simulink model "oc4_VarMass"  (R2026a)
settings: Solver=ode4  StartTime=0  StopTime=400  FixedStep=0.1  MaxStep=0.1  EnableMultiTasking=on
values from neighbouring files (symbols this model uses):
  simu = simulationClass()    [wecSimInputFile.m]
  waves = waveClass('regular')    [wecSimInputFile.m]
undefined symbols (not defined in the file or in its folder): body, constraint, X, Y, Z
libraries: nesl_utility x22, sm_lib x12, WECSim_Lib_Body_Elements x4, vrlib x1, matrix_library x1, WECSim_Lib_Constraints x1, WECSim_Lib_Frames x1
(part 2 of 3)

== system oc4_VarMass/Float/Hydrodynamic Body/Variable Hydrodynamics Control ==
  note: Developer note: When creating a new bus selector, it will only show the variables within hydroForce if they already exist in the workspace, which is inconventient. Copy this bus selector to more easily add calls to variables from hydroForce. This bus selector should already contains all variables in hydroForce which can then be selected, and extras deleted.
      |
      | Alternatively, open the bus selector block and use programmatic commands to set the output variables, e.g.
      | >> set_param(gcb, 'OutputSignals', 'storage.mass, volume');
  Bus Selector : BusSelector  Commented=on  OutputSignals=linearHydroRestCoef,storage,quadDrag,linearDamping,fExt,fExt.re,fExt.im,fExt.md,fAddedMass,fDamping,irkb,storage.mass,storage.inertia,storage.inertiaProducts,storage.fAddedMass,userDefinedFe,totDOF,fExt.dofGrd,fExt.dirGrd,fExt.wGrd,fExt.fEHRE,fExt.fEHIM,fExt.fEHMD
  Constant : Constant  Value=body.hydroForce  VectorParams1D=off  OutDataTypeStr=Bus: bus_body1_hydroForce
  From : From  Commented=on  GotoTag=body1_hydroForce
  Variable Hydrodynamics Subsystem : Subsystem  Variant=on  VariantControl=sv_b1_variableHydro  mask{body=body}
  tag scope: body1_hydroForce=global
  wires:
  From/1 -> Bus Selector/1
  Variable Hydrodynamics Subsystem/1(selected_hydroForce) -> [body1_hydroForce]
  Constant/1 -> Variable Hydrodynamics Subsystem/1(all_hydroForce)

== system oc4_VarMass/Float/Hydrodynamic Body/Wave Diffraction and Excitation Force Calculation ==
  note: The excitation force = F_wave * ramp function
  Time : Inport
  Displacement : Inport  Port=2
  WaveElv : Inport  Port=3
  Add : Sum  Inputs=+++
  Constant : Constant
  FexcInputs : Subsystem
  Less Than : RelationalOperator  Operator=<  OutDataTypeStr=boolean  RndMeth=Simplest  InputSameDT=off
  Linear Wave Excitation Force Variant Subsystem : Subsystem  Variant=on  VariantControl=sv_irregularWavesNonLinYaw_b1  mask{Nwave=waves(1)}
      mask prompts: Nwave "Wave Instance"
  Nonlinear FK Force Variant Subsystem : Subsystem  Variant=on
  Product : Product
  Ramp Function Time : Constant  Value=simu.rampTime
  Ramp function : Subsystem
  Second Order Excitation Force Variant Subsystem : Subsystem  Variant=on
  Switch : Switch  Criteria=u2 ~= 0  SaturateOnIntegerOverflow=off  InputSameDT=off
  F_Excitation : Outport  PortDimensions=body.dof
  wires:
  [body1_hydroForce] -> FexcInputs/4(body_hydroForce)
  FexcInputs/4(Out4) -> Second Order Excitation Force Variant Subsystem/2(body_hydroForce), Linear Wave Excitation Force Variant Subsystem/3(body_hydroForce)
  Second Order Excitation Force Variant Subsystem/1(Second Order Excitation) -> Add/3
  FexcInputs/1(Out1) -> Nonlinear FK Force Variant Subsystem/1(Time), Less Than/1, Ramp function/1(Time), Linear Wave Excitation Force Variant Subsystem/1(Time), Second Order Excitation Force Variant Subsystem/1(Time)
  FexcInputs/3(Out3) -> Nonlinear FK Force Variant Subsystem/3(WaveElv)
  WaveElv/1 -> FexcInputs/3(WaveElv)
  Displacement/1 -> FexcInputs/2(Displacement)
  Time/1 -> FexcInputs/1(Time)
  FexcInputs/2(Out2) -> Nonlinear FK Force Variant Subsystem/2(Displacement), Second Order Excitation Force Variant Subsystem/3(displacement), Linear Wave Excitation Force Variant Subsystem/2(Displacement)
  Constant/1 -> Switch/3
  Less Than/1 -> Switch/2
  Ramp function/1(R) -> Switch/1
  Ramp Function Time/1 -> Less Than/2
  Nonlinear FK Force Variant Subsystem/1(Nonlinear Excitation) -> Add/2
  Linear Wave Excitation Force Variant Subsystem/1(Linear Excitation) -> Add/1
  Product/1 -> F_Excitation/1  "F_Excitation"
  Add/1 -> Product/2  "F_wave"
  Switch/1 -> Product/1  "R"

== system oc4_VarMass/Float/Hydrodynamic Body/Wave Radiation Forces Calculation ==
  note: F_AddedMass = AM * a
  Velocity : Inport
  Acceleration : Inport  Port=2
  Bus Selector : BusSelector  OutputSignals=fAddedMass
  Product1 : Product  Multiplication=Matrix(*)
  SS CI and Constant-Damping-CoeVariant Subsystem : Subsystem  Variant=on
  F_RadiationDamping : Outport
  F_AddedMass : Outport  Port=2
  wires:
  Bus Selector/1 -> Product1/1  "<fAddedMass>"
  [body1_hydroForce] -> Bus Selector/1
  Acceleration/1 -> Product1/2
  SS CI and Constant-Damping-CoeVariant Subsystem/1(Out1) -> F_RadiationDamping/1  "F_RadiationDamping"
  Velocity/1 -> SS CI and Constant-Damping-CoeVariant Subsystem/1(velocity)
  Product1/1 -> F_AddedMass/1  "F_AddedMass"

== system oc4_VarMass/Float/Hydrodynamic Body/Yaw Force Transforms ==
  F_Excitation : Inport
  F_RadiationDamping : Inport  Port=2
  In2 : Inport  Port=3
  F_AddedMass : Inport  Port=4
  F_Restoring : Inport  Port=5
  Constant : Constant  Value=body.yaw.option
  Yaw Force Transforms : MATLAB Function  TreatAsAtomicUnit=on
  Out1 : Outport
  Out2 : Outport  Port=2
  Out3 : Outport  Port=3
  Out4 : Outport  Port=4
  wires:
  Yaw Force Transforms/1(F_Excitation) -> Out1/1
  Yaw Force Transforms/3(F_AddedMass) -> Out3/1
  Yaw Force Transforms/2(F_RadiationDamping) -> Out2/1
  F_RadiationDamping/1 -> Yaw Force Transforms/2(dispGlobal)
  F_AddedMass/1 -> Yaw Force Transforms/4(F_AddedMassLocal)
  Yaw Force Transforms/4(F_Restoring) -> Out4/1
  F_Excitation/1 -> Yaw Force Transforms/5(F_ExcitationLocal)
  In2/1 -> Yaw Force Transforms/3(F_RadiationDampingLocal)
  F_Restoring/1 -> Yaw Force Transforms/6(F_RestoringLocal)
  Constant/1 -> Yaw Force Transforms/1(yaw)

== system oc4_VarMass/Float/Hydrodynamic Body/Yaw Kinematic Transforms ==
  note: If simu.b2b == 0, no body to body interaction is used (noB2B)
      | If simu.b2b == 1, use body to body interaction (B2B)
  note: 1) Add Subsystem or Model blocks as valid variant choices.
      | 2) You cannot connect blocks at this level. At simulation, connectivity is automatically
      | determined, based on the active variant and port name matching.
  dispGlobal : Inport
  velGlobal : Inport  Port=2
  accGlobal : Inport  Port=3
  No B2B : Subsystem  VariantControl=sv_noB2B
  With B2B : Subsystem  VariantControl=sv_B2B
  dispLoc : Outport
  velLoc : Outport  Port=2
  accLoc : Outport  Port=3

== system oc4_VarMass/Float/Hydrodynamic Body/B2B Subsystem/B2B ==
  CrossCoupling : Subsystem  mask{body=body}
      mask prompts: body "Body Number"
      mask help: This is used to
      mask init:
      | %In the initialization tab we place the code modifying the block
      | 
      | cb = gcb;
      | % position of initial blocks
      | set_param([cb '/vel1'],'Position',[200 1*50 240 (1*50+30)])
      | set_param([cb '/Mux1'], 'Position',[375 40 380 90])
      | set_param([cb '/vel'], 'Position',[410 59 440 71])
      | set_param([cb '/acc1'],'Position',[600 1*50 640 (1*50+30)])
      | set_param([cb '/Mux2'], 'Position',[775 40 780 90])
      | set_param([cb '/acc'], 'Position',[810 59 840 71])
      | set_param([cb '/Transport Delay1'], 'Position', [650 1*50 690 (1*50+30)])
      | 
      | % add/delete lines & blocks
      | newInputs = 0;
      | numbodies = body.total;
      | iBod = 2;
      | while iBod < 100
      |     try 
      |         find_system([cb,'/vel',num2str(iBod)],'Type','Block');
      |         if iBod > numbodies
      |             %delete 'From' blocks and lines if bodynumber > total bodies
      |             delete_line(cb,['vel',num2str(iBod),'/1'],['Mux',num2str(1),'/',num2str(iBod)])
      |             delete_line(cb,['acc',num2str(iBod),'/1'],['Transport Delay',num2str(iBod),'/1'])
      |             delete_line(cb,['Transport Delay',num2str(iBod),'/1'],['Mux',num2str(2),'/',num2str(iBod)])
      |             delete_block([cb '/vel',num2str(iBod)])
      |             delete_block([cb '/acc',num2str(iBod)])
      |             delete_block([cb '/Transport Delay',num2str(iBod)])
      |         end
      |     catch
      |         %set number of outputs for 'Mux Creator' blocks 
      |         if newInputs==0
      |             set_param([cb,'/Mux1'],'Inputs',num2str(numbodies))
      |             set_param([cb,'/Mux2'],'Inputs',num2str(numbodies))
      |         end
      |         if iBod <= numbodies
      |             newInputs = newInputs + 1;
      |             %add velocity 'From' block
      |             add_block('simulink/Signal Routing/From', [cb,'/vel',num2str(iBod)],'MakeNameUnique', 'on',...
      |             'Position',[200 iBod*50 240 (iBod*50+30)], 'BackgroundColor','green')
      |             h=[cb,'/vel',num2str(iBod)];
      |             responseName=['vel' num2str(iBod)];
      |             set_param(h,'GotoTag',responseName);
      |             %add acceleration 'From' block
      |             add_block('simulink/Signal Routing/From', [cb,'/acc',num2str(iBod)],'MakeNameUnique', 'on',...
      |             'Position',[600 iBod*50 640 (iBod*50+30)], 'BackgroundColor','green')
      |             h=[cb,'/acc',num2str(iBod)];
      |             responseName=['acc' num2str(iBod)];
      |             set_param(h,'GotoTag',responseName);
      |             % add transport delay block 
      |             add_block('simulink/Continuous/Transport Delay', [cb,'/Transport Delay',num2str(iBod)],'MakeNameUnique', 'on',...
      |             'Position',[650 iBod*50 690 (iBod*50+30)])
      |             h=[cb,'/Transport Delay',num2str(iBod)];
      |             set_param(h,'DelayTime',num2str(10e-8));
      |             %add lines
      |             add_line(cb,['vel',num2str(iBod),'/1'],['Mux',num2str(1),'/',num2str(iBod)])
      |             add_line(cb,['acc',num2str(iBod),'/1'],['Transport Delay',num2str(iBod),'/1'])
      |             add_line(cb,['Transport Delay',num2str(iBod),'/1'],['Mux',num2str(2),'/',num2str(iBod)])
      |             
      |         else
      |             break
      |         end
      |     end
      |     iBod = iBod + 1;
      | end
      mask Callback body: %customsat_callback('input',gcb)
      mask DialogControl DescGroupVar Prompt: Coupling Block
      mask DialogControl DescTextVar Prompt: This block transfers the velocity and acceleration vectors between bodies allowing for the coupled hydrodynamic forces to be calculated.  This block should not be included if there is only one body or if the hydrodynamic coupling parameter is set to 'No' in the rigid body block.
  vel : Outport
  acc : Outport  Port=2
  wires:
  CrossCoupling/2(acc) -> acc/1
  CrossCoupling/1(vel) -> vel/1

== system oc4_VarMass/Float/Hydrodynamic Body/B2B Subsystem/noB2B ==
  vel_in : Inport
  acc_in : Inport  Port=2
  vel : Outport
  acc : Outport  Port=2
  wires:
  acc_in/1 -> acc/1
  vel_in/1 -> vel/1  "x"

== system oc4_VarMass/Float/Hydrodynamic Body/Hydrostatic Restoring Force Calculation/Linear and Nonlinear Restoring Force Variant Subsystem ==
  note: 1) Add Subsystem or Model blocks as valid variant choices.
      | 2) You cannot connect blocks at this level. At simulation, connectivity is automatically
      | determined, based on the active variant and port name matching.
  note: If simu.nlHydro == 0, use the linear force option.
      | If simu.nlHydro > 0, use the nonlinear force option.
  In1 : Inport
  In2 : Inport  Port=2
  Linear Hydrostatic Restoring Force : Subsystem  VariantControl=sv_b1_linearHydro
  Nonlinear Hydrostatic Restoring Force : Subsystem  VariantControl=sv_b1_nonlinearHydro
  Out1 : Outport

== system oc4_VarMass/Float/Hydrodynamic Body/Morison Element and Viscous Damping Force Calculation/Morison Element Variant Subsystem ==
  note: 1) Add Subsystem or Model blocks as valid variant choices.
      | 2) You cannot connect blocks at this level. At simulation, connectivity is automatically
      | determined, based on the active variant and port name matching.
  note: If body.morisonElement.option == 0, Morison element is off and the Morison force is 0
      | If body.morisonElement.option == 1 | 2, Morison element is on
  displacement : Inport
  velocity : Inport  Port=2
  acceleration : Inport  Port=3
  time : Inport  Port=4
  Morison Element Off : Subsystem  VariantControl=sv_b1_MEOff
  Morison Element On : Subsystem  Variant=on  VariantControl=sv_b1_MEOn
  morison_force : Outport

== system oc4_VarMass/Float/Hydrodynamic Body/Nonlinear Wave Elevation/Linear or Instantaneous Free Surface ==
  note: 1) Add Subsystem or Model blocks as valid variant choices.
      | 2) You cannot connect blocks at this level. At simulation, connectivity is automatically
      | determined, based on the active variant and port name matching.
  note: If simu.nlHydro < 2, use the mean water free surface.
      | If simu.nlHydro == 2, use the instantaneous water free surface
  In1 : Inport
  In2 : Inport  Port=2
  Instantaneous Water Free Surface : Subsystem  VariantControl=sv_b1_instFS
  Mean Water Free Surface : Subsystem  VariantControl=sv_b1_meanFS
  Out1 : Outport

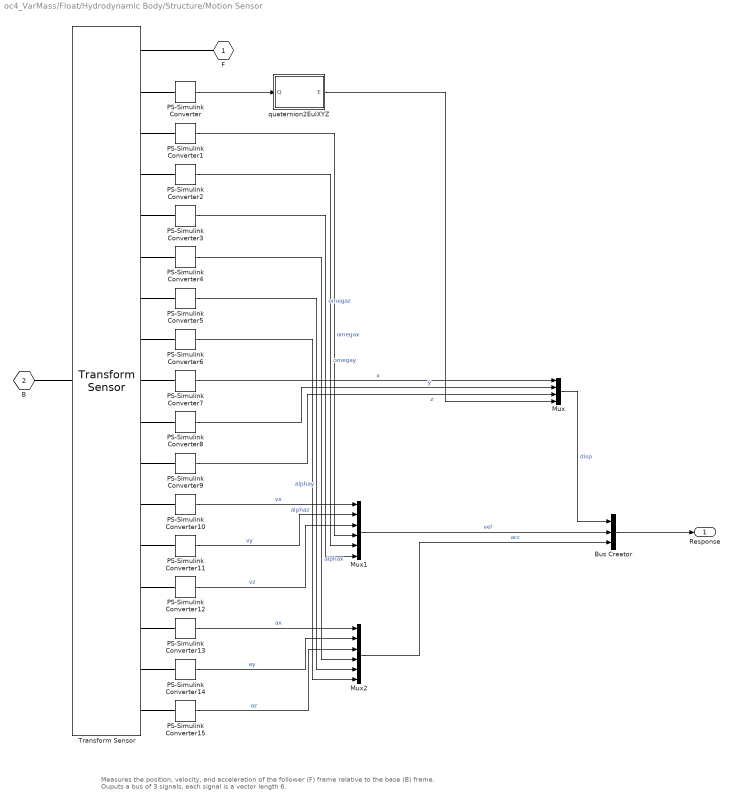
== system oc4_VarMass/Float/Hydrodynamic Body/Structure/Motion Sensor ==
  note: Measures the position, velocity, and acceleration of the follower (F) frame relative to the base (B) frame.
      | Ouputs a bus of 3 signals, each signal is a vector length 6.
  Bus Creator : BusCreator  Inputs=3
  Mux : Mux
  Mux1 : Mux  Inputs=6
  Mux2 : Mux  Inputs=6
  PS-Simulink Converter{,1..15} (16 alike) : nesl_utility/PS-Simulink Converter  PhysicalDomain=network_engine_domain  SubClassName=ps_output  LeftPortType=input  RightPortType=output  PseudoPeriodic=off  Frequencies=[]  VectorFormat=1-D array  Unit=1  AffineConversion=off
  Transform Sensor : sm_lib/Frames and Transforms/Transform Sensor  MeasurementFrame=World  RotationSequence=XYX  SenseAngle=off  SenseAxis=off  SenseQ=on  SenseR=off  SenseRotationSequence=off  SenseOmegaX=on  SenseOmegaY=on  SenseOmegaZ=on  SenseOmega=off  SenseQDot=off  SenseRDot=off  SenseRotationSequenceDot=off  SenseAlphaX=on  SenseAlphaY=on  SenseAlphaZ=on  SenseAlpha=off  SenseQDDot=off  SenseRDDot=off  SenseX=on  SenseY=on  SenseZ=on  SenseXYZ=off  SenseRad=off  SenseAzim=off  SenseDist=off  SenseInc=off  SenseXDot=on  SenseYDot=on  SenseZDot=on  SenseXYZDot=off  SenseRadDot=off  SenseAzimDot=off  SenseDistDot=off  SenseIncDot=off  SenseXDDot=on  SenseYDDot=on  SenseZDDot=on  SenseXYZDDot=off  SenseRadDDot=off  SenseAzimDDot=off  SenseDistDDot=off  SenseIncDDot=off
  quaternion2EulXYZ : MATLAB Function  TreatAsAtomicUnit=on
  F : PMIOPort  Side=Right
  B : PMIOPort  Port=2  Side=Left
  Response : Outport
  wires:
  PS-Simulink Converter/1 -> quaternion2EulXYZ/1(Q)
  quaternion2EulXYZ/1(E) -> Mux/4
  PS-Simulink Converter4/1 -> Mux2/4  "alphax"
  PS-Simulink Converter10/1 -> Mux1/1  "vx"
  PS-Simulink Converter12/1 -> Mux1/3  "vz"
  PS-Simulink Converter13/1 -> Mux2/1  "ax"
  PS-Simulink Converter14/1 -> Mux2/2  "ay"
  Mux/1 -> Bus Creator/1  "disp"
  Mux1/1 -> Bus Creator/2  "vel"
  Mux2/1 -> Bus Creator/3  "acc"
  PS-Simulink Converter7/1 -> Mux/1  "x"
  PS-Simulink Converter8/1 -> Mux/2  "y"
  PS-Simulink Converter9/1 -> Mux/3  "z"
  PS-Simulink Converter5/1 -> Mux2/5  "alphay"
  PS-Simulink Converter6/1 -> Mux2/6  "alphaz"
  PS-Simulink Converter1/1 -> Mux1/4  "omegax"
  PS-Simulink Converter2/1 -> Mux1/5  "omegay"
  PS-Simulink Converter11/1 -> Mux1/2  "vy"
  PS-Simulink Converter3/1 -> Mux1/6  "omegaz"
  PS-Simulink Converter15/1 -> Mux2/3  "az"
  Bus Creator/1 -> Response/1
  connections:
  Transform Sensor/RConn16 -- PS-Simulink Converter14/LConn1
  PS-Simulink Converter13/LConn1 -- Transform Sensor/RConn15
  PS-Simulink Converter12/LConn1 -- Transform Sensor/RConn14
  Transform Sensor/RConn13 -- PS-Simulink Converter11/LConn1
  PS-Simulink Converter10/LConn1 -- Transform Sensor/RConn12
  PS-Simulink Converter9/LConn1 -- Transform Sensor/RConn11
  Transform Sensor/RConn10 -- PS-Simulink Converter8/LConn1
  PS-Simulink Converter7/LConn1 -- Transform Sensor/RConn9
  Transform Sensor/RConn8 -- PS-Simulink Converter6/LConn1
  PS-Simulink Converter5/LConn1 -- Transform Sensor/RConn7
  Transform Sensor/RConn6 -- PS-Simulink Converter4/LConn1
  PS-Simulink Converter3/LConn1 -- Transform Sensor/RConn5
  Transform Sensor/RConn4 -- PS-Simulink Converter2/LConn1
  PS-Simulink Converter1/LConn1 -- Transform Sensor/RConn3
  Transform Sensor/RConn2 -- PS-Simulink Converter/LConn1
  PS-Simulink Converter15/LConn1 -- Transform Sensor/RConn17
  Transform Sensor/RConn1 -- F/RConn1
  B/RConn1 -- Transform Sensor/LConn1

== system oc4_VarMass/Float/Hydrodynamic Body/Variable Hydrodynamics Control/Variable Hydrodynamics Subsystem ==
  note: 1) Add Subsystem or Model blocks as valid variant choices.
      | 2) You cannot connect blocks at this level. At simulation, connectivity is automatically
      | determined, based on the active variant and port name matching.
  all_hydroForce : Inport
  noVariableHydro : Subsystem  VariantControl=sv_b1_noVariableHydro
  variableHydro : Subsystem  VariantControl=sv_b1_variableHydro  mask{body=body}
      mask prompts: body "Body Number:"
      mask init:
      | hydroForceElements = fields(body.hydroForce);
      | 
      | nElements = length(hydroForceElements);
      | elementString = hydroForceElements{1};
      | if nElements > 1
      |     for i=2:nElements
      |         elementString = [elementString ', ' hydroForceElements{i}]; 
      |     end
      | end
      | 
      | % Update bus signals with the name of hydroForce elements (hf1, hf2, etc)
      | h = [gcb '/Bus Selector'];
      | set_param(h, 'OutputSignals', elementString);
      | 
      | % Update number of switch inputs
      | h = [gcb '/Multiport Switch'];
      | set_param(h, 'Inputs', num2str(nElements));
      | 
      | % Connect bus outputs and switch inputs
      | for i = 1:nElements
      |     try
      |         add_line(gcb, ...
      |             ['Bus Selector/' num2str(i)], ...
      |             ['Multiport Switch/' num2str(i+1)],...
      |             'autorouting','on');
      |     catch
      |     end
      | end
      | 
      | % Connect the initial case (default hydroForce) to the end of the multiport switch (default case)
      | hydroForceIndexInitial = body.variableHydro.hydroForceIndexInitial;
      | try
      |     add_line(gcb, ...
      |         ['Bus Selector/' num2str(hydroForceIndexInitial)], ...
      |         ['Multiport Switch/' num2str(nElements+2)],...
      |         'autorouting','on');
      | catch
      | end
  selected_hydroForce : Outport

== system oc4_VarMass/Float/Hydrodynamic Body/Wave Diffraction and Excitation Force Calculation/FexcInputs ==
  Time : Inport
  Displacement : Inport  Port=2
  WaveElv : Inport  Port=3
  body_hydroForce : Inport  Port=4
  Out1 : Outport
  Out2 : Outport  Port=2
  Out3 : Outport  Port=3
  Out4 : Outport  Port=4
  wires:
  body_hydroForce/1 -> Out4/1
  Displacement/1 -> Out2/1
  Time/1 -> Out1/1
  WaveElv/1 -> Out3/1

== system oc4_VarMass/Float/Hydrodynamic Body/Wave Diffraction and Excitation Force Calculation/Linear Wave Excitation Force Variant Subsystem ==
  note: 1) Add Subsystem or Model blocks as valid variant choices.
      | 2) You cannot connect blocks at this level. At simulation, connectivity is automatically
      | determined, based on the active variant and port name matching.
  note: No wave includes wave.type == 'noWave' or 'noWaveCIC'
      | Regular wave includes wave.type == 'regular' or 'regularCIC'
      | Irregular wave includes wave.type == 'irregular' or 'spectrumImport'
  Time : Inport
  Displacement : Inport  Port=2
  body_hydroForce : Inport  Port=3
  Irregular Wave Excitation Force : Subsystem  VariantControl=sv_irregularWaves_b1
  Irregular Wave NonLinearYaw : Subsystem  VariantControl=sv_irregularWavesYaw_b1
  Irregular Wave Full Direction : Subsystem  VariantControl=sv_fullDirIrregularWaves_b1
  No Wave Excitation Force : Subsystem  VariantControl=sv_noWave
  Regular Wave Excitation Force : Subsystem  VariantControl=sv_regularWaves_b1
  Regular Wave NonLinear Yaw : Subsystem  VariantControl=sv_regularWavesYaw_b1
  User Defined Wave Excitation Force : Subsystem  VariantControl=sv_udfWaves
  Linear Excitation : Outport

== system oc4_VarMass/Float/Hydrodynamic Body/Wave Diffraction and Excitation Force Calculation/Nonlinear FK Force Variant Subsystem ==
  note: 1) Add Subsystem or Model blocks as valid variant choices.
      | 2) You cannot connect blocks at this level. At simulation, connectivity is automatically
      | determined, based on the active variant and port name matching.
  note: If simu.nlHydro == 0, use No Nonlinear FroudeKrylov force option (nonlinear force is zero),
      | If simu.nlHydro > 0, use the Nonlinear FroudeKrylov force option,
  Time : Inport
  Displacement : Inport  Port=2
  WaveElv : Inport  Port=3
  No Nonlinear FroudeKrylov Force : Subsystem  VariantControl=sv_b1_linearHydro
  With Nonlinear FroudeKrylov Force : Subsystem  TreatAsAtomicUnit=on  SystemSampleTime=simu.nonlinearDt  VariantControl=sv_b1_nonlinearHydro
  Nonlinear Excitation : Outport

== system oc4_VarMass/Float/Hydrodynamic Body/Wave Diffraction and Excitation Force Calculation/Ramp function ==
  note: The ramp function R, is a smooth function:
      | R = (sin(3*pi/2 + pi * t/Tr) + 1)/2 from t=0 to t=Tr
  Time : Inport
  Add1 : Sum
  Add2 : Sum
  Constant1 : Constant  Value=1/2
  Constant2 : Constant
  Constant3 : Constant  Value=3*pi/2
  Constant4 : Constant  Value=pi
  Divide : Product  Inputs=*/
  Product1 : Product
  Product2 : Product
  Ramp Time : Constant  Value=simu.rampTime
  Sine Wave Function : Sin  TimeSource=Use external signal  SampleTime=0
  R : Outport
  wires:
  Product1/1 -> R/1
  Constant2/1 -> Add1/1
  Constant3/1 -> Add2/2  "phase"
  Ramp Time/1 -> Divide/2  "t_ramp"
  Divide/1 -> Product2/2  "frequency"
  Add1/1 -> Product1/1
  Constant4/1 -> Divide/1
  Add2/1 -> Sine Wave Function/1
  Product2/1 -> Add2/1
  Time/1 -> Product2/1
  Sine Wave Function/1 -> Add1/2
  Constant1/1 -> Product1/2

== system oc4_VarMass/Float/Hydrodynamic Body/Wave Diffraction and Excitation Force Calculation/Second Order Excitation Force Variant Subsystem ==
  note: 1) Add Subsystem or Model blocks as valid variant choices.
      | 2) You cannot connect blocks at this level. At simulation, connectivity is automatically
      | determined, based on the active variant and port name matching.
  Time : Inport
  body_hydroForce : Inport  Port=2
  displacement : Inport  Port=3
  No Second Order Excitation Force : Subsystem  VariantControl=sv_b1_noSecondOrderExt
  With Second Order Excitation Force : Subsystem  VariantControl=sv_b1_secondOrderExt
  Second Order Excitation : Outport

== system oc4_VarMass/Float/Hydrodynamic Body/Wave Radiation Forces Calculation/SS CI and Constant-Damping-CoeVariant Subsystem ==
  note: 1) Add Subsystem or Model blocks as valid variant choices.
      | 2) You cannot connect blocks at this level. At simulation, connectivity is automatically
      | determined, based on the active variant and port name matching.
  note: If the wave type is 'noWave' or 'regular' use constant coefficients.
      | If another wave type and simu.Calc ~= 1, use convolution integral calculation
      | If another wave type and simu.Calc == 1, use the state space calculation
      | If another wave type and simu.FIR == 1, use the FIR filter calculation
  velocity : Inport
  Constant Coefficients : Subsystem  VariantControl=sv_constantCoeff
  Convolution Integral Calculation : Subsystem  VariantControl=sv_convolution
  FIR Filter Calculation : Subsystem  VariantControl=sv_FIR
  "State-Space Calculation " : Subsystem  VariantControl=sv_stateSpace
  Out1 : Outport

== system oc4_VarMass/Float/Hydrodynamic Body/Yaw Kinematic Transforms/No B2B ==
  note: If body.yaw.option == 1, interpolate the BEM coefficients to account for the effective change in the incoming wave direction.
  dispGlobal : Inport
  velGlobal : Inport  Port=2
  accGlobal : Inport  Port=3
  Constant : Constant  Value=body.yaw.option
  Yaw Kinematic Transforms : MATLAB Function  TreatAsAtomicUnit=on
  dispLoc : Outport
  velLoc : Outport  Port=2
  accLoc : Outport  Port=3
  wires:
  Yaw Kinematic Transforms/3(accLoc) -> accLoc/1
  Yaw Kinematic Transforms/1(dispLoc) -> dispLoc/1
  Yaw Kinematic Transforms/2(velLoc) -> velLoc/1
  Constant/1 -> Yaw Kinematic Transforms/1(yaw)
  accGlobal/1 -> Yaw Kinematic Transforms/4(accGlobal)
  velGlobal/1 -> Yaw Kinematic Transforms/3(velGlobal)
  dispGlobal/1 -> Yaw Kinematic Transforms/2(dispGlobal)

== system oc4_VarMass/Float/Hydrodynamic Body/Yaw Kinematic Transforms/With B2B ==
  note: If body.yaw.option == 1, interpolate the BEM coefficients to account for the effective change in the incoming wave direction.
  dispGlobal : Inport
  velGlobal : Inport  Port=2
  accGlobal : Inport  Port=3
  Constant : Constant  Value=body.yaw.option
  Yaw Kinematic Transforms : MATLAB Function  TreatAsAtomicUnit=on
  dispLoc : Outport
  velLoc : Outport  Port=2
  accLoc : Outport  Port=3
  wires:
  accGlobal/1 -> Yaw Kinematic Transforms/4(accGlobal)
  velGlobal/1 -> Yaw Kinematic Transforms/3(velGlobal)
  dispGlobal/1 -> Yaw Kinematic Transforms/2(dispGlobal)
  Yaw Kinematic Transforms/3(accLoc) -> accLoc/1
  Yaw Kinematic Transforms/2(velLoc) -> velLoc/1
  Yaw Kinematic Transforms/1(dispLoc) -> dispLoc/1
  Constant/1 -> Yaw Kinematic Transforms/1(yaw)

== system oc4_VarMass/Float/Hydrodynamic Body/B2B Subsystem/B2B/CrossCoupling ==
  note: CrossCoupling block is updated by its mask initialization, which is only called on when a simulation is run. 'From' blocks are automatically created and connected based on the number of bodies in the simulation.
  Mux1 : Mux  Inputs=2
  Mux2 : Mux  Inputs=2
  Transport Delay1 : TransportDelay  DelayTime=10e-8
  Transport Delay2 : TransportDelay  DelayTime=1e-07
  vel : Outport
  acc : Outport  Port=2
  wires:
  Transport Delay2/1 -> Mux2/2
  [acc2] -> Transport Delay2/1
  [vel2] -> Mux1/2
  Transport Delay1/1 -> Mux2/1
  Mux2/1 -> acc/1
  [acc1] -> Transport Delay1/1
  Mux1/1 -> vel/1
  [vel1] -> Mux1/1

== system oc4_VarMass/Float/Hydrodynamic Body/Hydrostatic Restoring Force Calculation/Linear and Nonlinear Restoring Force Variant Subsystem/Linear Hydrostatic Restoring Force ==
  note: The total hydrostatic restoring force is due to a linear stiffness, the vertical buoyancy force (gravity - buoyancy) and a rotational buoyancy force if the center of gravity is not aligned with the center of buoyancy.
      |
      | F_restoring = F_linearRestoringStiffness + F_NetBuoyancy
      |
      | F_linear restoring = hydrostatic restoring coefficient * displacement
      | F_NetBuoyancy = F_gravity - F_buoyancy + F_rotational_buoyancy
      |
      | F_rotational_buoyancy = (cb-cg) x F_buoyancy
      | F_buoyancy = rho*g*V_0
      | F_gravity = m*g
  In1 : Inport
  Add : Sum
  Bus Selector : BusSelector  OutputSignals=mass,volume,centerBuoyancy,linearHydroRestCoef
  Net Buoyancy Force : Subsystem
  Product2 : Product  Multiplication=Matrix(*)
  Out1 : Outport
  wires:
  Bus Selector/1 -> Net Buoyancy Force/1(Body Mass)  "<mass>"
  Bus Selector/2 -> Net Buoyancy Force/2(Volume)  "<volume>"
  Bus Selector/3 -> Net Buoyancy Force/3(Center of Buoyancy)  "<centerBuoyancy>"
  [body1_hydroForce] -> Bus Selector/1
  Net Buoyancy Force/1(F_NetBuoyancy) -> Add/1  "Net buoyancy force"
  Product2/1 -> Add/2  "Linear Restoring Force"
  Add/1 -> Out1/1  "F_Restoring"
  Bus Selector/4 -> Product2/1  "<linearHydroRestCoef>"
  In1/1 -> Product2/2  "x"

== system oc4_VarMass/Float/Hydrodynamic Body/Hydrostatic Restoring Force Calculation/Linear and Nonlinear Restoring Force Variant Subsystem/Nonlinear Hydrostatic Restoring Force ==
  In1 : Inport
  In2 : Inport  Port=2
  Bus Selector : BusSelector  OutputSignals=mass
  Center of Gravity : Constant  Value=body.centerGravity
  Gravity2 : Constant  Value=simu.gravity
  Rate Transition : RateTransition
  Rate Transition1 : RateTransition
  Restoring Forces : MATLAB Function  TreatAsAtomicUnit=on  SystemSampleTime=simu.nonlinearDt
  STL areas : Constant  Value=body.geometry.area
  STL centers : Constant  Value=body.geometry.center
  STL normal vectors : Constant  Value=body.geometry.norm
  To Workspace1 : ToWorkspace  VariableName=body1_hspressure_out  SaveFormat=Structure With Time  SampleTime=-1
      settings: Decimation=round(simu.dtOut/simu.dt,0)
  Water Density1 : Constant  Value=simu.rho
  Out1 : Outport
  wires:
  [body1_hydroForce] -> Bus Selector/1
  Rate Transition/1 -> Out1/1
  Restoring Forces/1(f) -> Rate Transition/1
  Rate Transition1/1 -> To Workspace1/1
  Restoring Forces/2(p) -> Rate Transition1/1
  Bus Selector/1 -> Restoring Forces/9(mass)  "<mass>"
  STL areas/1 -> Restoring Forces/5(area)
  In2/1 -> Restoring Forces/2(elv)
  STL centers/1 -> Restoring Forces/3(center)
  STL normal vectors/1 -> Restoring Forces/4(tnorm)
  Water Density1/1 -> Restoring Forces/6(rho)
  Gravity2/1 -> Restoring Forces/7(g)  "g"
  Center of Gravity/1 -> Restoring Forces/8(cg)
  In1/1 -> Restoring Forces/1(x)

== system oc4_VarMass/Float/Hydrodynamic Body/Morison Element and Viscous Damping Force Calculation/Morison Element Variant Subsystem/Morison Element Off ==
  Constant : Constant  Value=zeros(1,body.dof)
  morison_force : Outport
  wires:
  Constant/1 -> morison_force/1

== system oc4_VarMass/Float/Hydrodynamic Body/Morison Element and Viscous Damping Force Calculation/Morison Element Variant Subsystem/Morison Element On ==
  note: 1) Add Subsystem or Model blocks as valid variant choices.
      | 2) You cannot connect blocks at this level. At simulation, connectivity is automatically
      | determined, based on the active variant and port name matching.
  note: Chooses the appropriate Morison element variant dependent on the wave type. Note that if passive yaw is used, no block is chosen.
      |
      | If wave.type == 'noWave' | 'noWaveCIC' use No Wave Morison element
      | If wave.type == 'regularWave' | 'regularWaveCIC' use Regular Wave Morison element
      | If wave.type == 'irregularWave' or 'spectrumImport' use Irregular Wave Morison element
  displacement : Inport
  velocity : Inport  Port=2
  acceleration : Inport  Port=3
  time : Inport  Port=4
  Irregular Wave Morison Force : Subsystem  TreatAsAtomicUnit=on  SystemSampleTime=simu.morisonDt  VariantControl=sv_irregularWaves_b1
  No Wave Morison Force : Subsystem  VariantControl=sv_noWave
  Regular Wave Morison Force : Subsystem  TreatAsAtomicUnit=on  SystemSampleTime=simu.morisonDt  VariantControl=sv_regularWaves_b1
  morison_force : Outport

== system oc4_VarMass/Float/Hydrodynamic Body/Nonlinear Wave Elevation/Linear or Instantaneous Free Surface/Instantaneous Water Free Surface ==
  note: Calculate the instantaneous wave elevation for the nonlinear hydrodynamics options.
  In1 : Inport
  In2 : Inport  Port=2
  Center of Gravity : Constant  Value=body.centerGravity
  Frequency Spacing : Constant  Value=waves.dOmega
  Instantaneous FS : MATLAB Function  TreatAsAtomicUnit=on
  Ramp Time : Constant  Value=simu.rampTime
  STL Centers : Constant  Value=body.geometry.center
  Wave Amplitude : Constant  Value=waves.amplitude
  Wave Direction : Constant  Value=waves.direction
  Wave Frequency : Constant  Value=waves.omega
  Wave Number : Constant  Value=waves.wavenumber
  Wave Random Phase : Constant  Value=waves.phase
  Wave Spread : Constant  Value=waves.spread
  Wave Type Number : Constant  Value=waves.typeNum
  Out1 : Outport
  wires:
  Wave Spread/1 -> Instantaneous FS/13(spread)
  Wave Amplitude/1 -> Instantaneous FS/4(AH)
  Wave Direction/1 -> Instantaneous FS/12(waveDir)
  In1/1 -> Instantaneous FS/1(x)
  In2/1 -> Instantaneous FS/9(t)
  Frequency Spacing/1 -> Instantaneous FS/6(dw)
  Wave Random Phase/1 -> Instantaneous FS/11(phaseRand)
  Ramp Time/1 -> Instantaneous FS/10(rampT)
  Wave Type Number/1 -> Instantaneous FS/8(typeNum)
  Wave Frequency/1 -> Instantaneous FS/5(w)
  Wave Number/1 -> Instantaneous FS/7(k)
  Center of Gravity/1 -> Instantaneous FS/3(cg)
  STL Centers/1 -> Instantaneous FS/2(center)
  Instantaneous FS/1(f) -> Out1/1

== system oc4_VarMass/Float/Hydrodynamic Body/Nonlinear Wave Elevation/Linear or Instantaneous Free Surface/Mean Water Free Surface ==
  note: The mean water surface is always zero.
  zero : Constant  Value=0
  Out1 : Outport
  wires:
  zero/1 -> Out1/1

== system oc4_VarMass/Float/Hydrodynamic Body/Variable Hydrodynamics Control/Variable Hydrodynamics Subsystem/noVariableHydro ==
  all_hydroForce : Inport
  Bus Selector : BusSelector  OutputSignals=hf1
  selected_hydroForce : Outport
  wires:
  all_hydroForce/1 -> Bus Selector/1  "x"
  Bus Selector/1 -> selected_hydroForce/1  "<hf1>"

== system oc4_VarMass/Float/Hydrodynamic Body/Variable Hydrodynamics Control/Variable Hydrodynamics Subsystem/variableHydro ==
  all_hydroForce : Inport
  Bus Selector : BusSelector  OutputSignals=hf1,hf2,hf3,hf4,hf5,hf6,hf7,hf8,hf9,hf10,hf11,hf12,hf13,hf14,hf15,hf16,hf17,hf18,hf19,hf20,hf21,hf22,hf23,hf24,hf25,hf26,hf27,hf28,hf29,hf30,hf31,hf32,hf33,hf34,hf35,hf36,hf37,hf38,hf39,hf40,hf41,hf42,hf43,hf44,hf45,hf46,hf47,hf48,hf49,hf50,hf51,hf52,hf53,hf54,hf55,hf56,hf57,hf58,hf59,hf60,hf61,hf62,hf63,hf64,hf65,hf66,hf67,hf68,hf69,hf70,hf71,hf72,hf73,hf74,hf75,hf76,hf77,hf78,hf79,hf80,hf81
  Multiport Switch : MultiPortSwitch  Inputs=81  DataPortForDefault=Additional data port  DiagnosticForDefault=Warning  OutDataTypeStr=Inherit: Same as first data input  RndMeth=Round  SaturateOnIntegerOverflow=off  InputSameDT=off
      settings: LockScale=on
  To Workspace : ToWorkspace  VariableName=body1_hydroForceIndex  SaveFormat=Structure With Time  SampleTime=simu.dtOut
  selected_hydroForce : Outport
  wires:
  Bus Selector/1 -> Multiport Switch/2, Multiport Switch/83  "<hf1>"
  Multiport Switch/1 -> selected_hydroForce/1
  [body1_hydroForceIndex] -> Multiport Switch/1, To Workspace/1
  all_hydroForce/1 -> Bus Selector/1
  Bus Selector/2 -> Multiport Switch/3  "<hf2>"
  Bus Selector/3 -> Multiport Switch/4  "<hf3>"
  Bus Selector/4 -> Multiport Switch/5  "<hf4>"
  Bus Selector/5 -> Multiport Switch/6  "<hf5>"
  Bus Selector/6 -> Multiport Switch/7  "<hf6>"
  Bus Selector/7 -> Multiport Switch/8  "<hf7>"
  Bus Selector/8 -> Multiport Switch/9  "<hf8>"
  Bus Selector/9 -> Multiport Switch/10  "<hf9>"
  Bus Selector/10 -> Multiport Switch/11  "<hf10>"
  Bus Selector/11 -> Multiport Switch/12  "<hf11>"
  Bus Selector/12 -> Multiport Switch/13  "<hf12>"
  Bus Selector/13 -> Multiport Switch/14  "<hf13>"
  Bus Selector/14 -> Multiport Switch/15  "<hf14>"
  Bus Selector/15 -> Multiport Switch/16  "<hf15>"
  Bus Selector/16 -> Multiport Switch/17  "<hf16>"
  Bus Selector/17 -> Multiport Switch/18  "<hf17>"
  Bus Selector/18 -> Multiport Switch/19  "<hf18>"
  Bus Selector/19 -> Multiport Switch/20  "<hf19>"
  Bus Selector/20 -> Multiport Switch/21  "<hf20>"
  Bus Selector/21 -> Multiport Switch/22  "<hf21>"
  Bus Selector/22 -> Multiport Switch/23  "<hf22>"
  Bus Selector/23 -> Multiport Switch/24  "<hf23>"
  Bus Selector/24 -> Multiport Switch/25  "<hf24>"
  Bus Selector/25 -> Multiport Switch/26  "<hf25>"
  Bus Selector/26 -> Multiport Switch/27  "<hf26>"
  Bus Selector/27 -> Multiport Switch/28  "<hf27>"
  Bus Selector/28 -> Multiport Switch/29  "<hf28>"
  Bus Selector/29 -> Multiport Switch/30  "<hf29>"
  Bus Selector/30 -> Multiport Switch/31  "<hf30>"
  Bus Selector/31 -> Multiport Switch/32  "<hf31>"
  Bus Selector/32 -> Multiport Switch/33  "<hf32>"
  Bus Selector/33 -> Multiport Switch/34  "<hf33>"
  Bus Selector/34 -> Multiport Switch/35  "<hf34>"
  Bus Selector/35 -> Multiport Switch/36  "<hf35>"
  Bus Selector/36 -> Multiport Switch/37  "<hf36>"
  Bus Selector/37 -> Multiport Switch/38  "<hf37>"
  Bus Selector/38 -> Multiport Switch/39  "<hf38>"
  Bus Selector/39 -> Multiport Switch/40  "<hf39>"
  Bus Selector/40 -> Multiport Switch/41  "<hf40>"
  Bus Selector/41 -> Multiport Switch/42  "<hf41>"
  Bus Selector/42 -> Multiport Switch/43  "<hf42>"
  Bus Selector/43 -> Multiport Switch/44  "<hf43>"
  Bus Selector/44 -> Multiport Switch/45  "<hf44>"
  Bus Selector/45 -> Multiport Switch/46  "<hf45>"
  Bus Selector/46 -> Multiport Switch/47  "<hf46>"
  Bus Selector/47 -> Multiport Switch/48  "<hf47>"
  Bus Selector/48 -> Multiport Switch/49  "<hf48>"
  Bus Selector/49 -> Multiport Switch/50  "<hf49>"
  Bus Selector/50 -> Multiport Switch/51  "<hf50>"
  Bus Selector/51 -> Multiport Switch/52  "<hf51>"
  Bus Selector/52 -> Multiport Switch/53  "<hf52>"
  Bus Selector/53 -> Multiport Switch/54  "<hf53>"
  Bus Selector/54 -> Multiport Switch/55  "<hf54>"
  Bus Selector/55 -> Multiport Switch/56  "<hf55>"
  Bus Selector/56 -> Multiport Switch/57  "<hf56>"
  Bus Selector/57 -> Multiport Switch/58  "<hf57>"
  Bus Selector/58 -> Multiport Switch/59  "<hf58>"
  Bus Selector/59 -> Multiport Switch/60  "<hf59>"
  Bus Selector/60 -> Multiport Switch/61  "<hf60>"
  Bus Selector/61 -> Multiport Switch/62  "<hf61>"
  Bus Selector/62 -> Multiport Switch/63  "<hf62>"
  Bus Selector/63 -> Multiport Switch/64  "<hf63>"
  Bus Selector/64 -> Multiport Switch/65  "<hf64>"
  Bus Selector/65 -> Multiport Switch/66  "<hf65>"
  Bus Selector/66 -> Multiport Switch/67  "<hf66>"
  Bus Selector/67 -> Multiport Switch/68  "<hf67>"
  Bus Selector/68 -> Multiport Switch/69  "<hf68>"
  Bus Selector/69 -> Multiport Switch/70  "<hf69>"
  Bus Selector/70 -> Multiport Switch/71  "<hf70>"
  Bus Selector/71 -> Multiport Switch/72  "<hf71>"
  Bus Selector/72 -> Multiport Switch/73  "<hf72>"
  Bus Selector/73 -> Multiport Switch/74  "<hf73>"
  Bus Selector/74 -> Multiport Switch/75  "<hf74>"
  Bus Selector/75 -> Multiport Switch/76  "<hf75>"
  Bus Selector/76 -> Multiport Switch/77  "<hf76>"
  Bus Selector/77 -> Multiport Switch/78  "<hf77>"
  Bus Selector/78 -> Multiport Switch/79  "<hf78>"
  Bus Selector/79 -> Multiport Switch/80  "<hf79>"
  Bus Selector/80 -> Multiport Switch/81  "<hf80>"
  Bus Selector/81 -> Multiport Switch/82  "<hf81>"

== system oc4_VarMass/Float/Hydrodynamic Body/Wave Diffraction and Excitation Force Calculation/Linear Wave Excitation Force Variant Subsystem/Irregular Wave Excitation Force ==
  note: Calculates the wave force, F_wave, for the case of Irregular Waves.
      |
      | The total force is the combination of the real excitation force, imaginary excitation force, and real part of the mean drift force (fExt.md)
      |
      | F_wave =   sum(A * cos(w * t) * Re{Fext(i)}
      |                            -  A * sin(w * t) * Im{Fext(i)}
      |                            + A * Re(Fext.md(i))
      |                            )
      |
      | where i = each frequency bin
  Time : Inport
  Displacement : Inport  Port=2
  body_hydroForce : Inport  Port=3
  Bus Selector : BusSelector  OutputSignals=fExt.re,fExt.im,fExt.md
  Displacement Phase Enable1 : Constant  Value=body.largeXYDisplacement.option
  Frequency Spacing Delta Omega : Constant  Value=Nwave.dOmega  VectorParams1D=off
  MATLAB Function : MATLAB Function  TreatAsAtomicUnit=on
  MATLAB Function2 : MATLAB Function  TreatAsAtomicUnit=on
  Random Phase : Constant  Value=Nwave.phase  VectorParams1D=off
  Selector : Selector  IndexOptions=Index vector (dialog)  Indices=[1 2]  OutputSizes=1
  Sum : Sum  Inputs=|++
  Wave Frequency : Constant  Value=Nwave.omega  VectorParams1D=off
  Wave Frequency1 : Constant  Value=Nwave.omega  VectorParams1D=off
  Wave Number1 : Constant  Value=Nwave.wavenumber
  Wave Spectrum : Constant  Value=Nwave.amplitude  VectorParams1D=off
  Wave direction spread : Constant  Value=Nwave.spread  VectorParams1D=off
  Wave direction1 : Constant  Value=Nwave.direction  VectorParams1D=off
  Linear Excitation : Outport
  wires:
  body_hydroForce/1 -> Bus Selector/1
  Bus Selector/1 -> MATLAB Function/3(fExtRE)  "<re>"
  Wave direction1/1 -> MATLAB Function2/5(direction), MATLAB Function/8(WaveDir)
  Wave Number1/1 -> MATLAB Function2/4(wavenumber)
  Displacement/1 -> Selector/1  "t"
  Selector/1 -> MATLAB Function2/1(disp)
  Displacement Phase Enable1/1 -> MATLAB Function2/2(enable)
  Wave Frequency1/1 -> MATLAB Function2/3(frequency)
  Random Phase/1 -> Sum/1
  Sum/1 -> MATLAB Function/5(phaseRand)
  MATLAB Function2/1(dispPhase) -> Sum/2
  Bus Selector/3 -> MATLAB Function/10(fExtMD)  "<md>"
  Wave direction spread/1 -> MATLAB Function/9(spread)
  Frequency Spacing Delta Omega/1 -> MATLAB Function/6(dw)
  Time/1 -> MATLAB Function/7(time)
  Wave Spectrum/1 -> MATLAB Function/1(A)
  Bus Selector/2 -> MATLAB Function/4(fExtIM)  "<im>"
  Wave Frequency/1 -> MATLAB Function/2(w)
  MATLAB Function/1(Fext) -> Linear Excitation/1

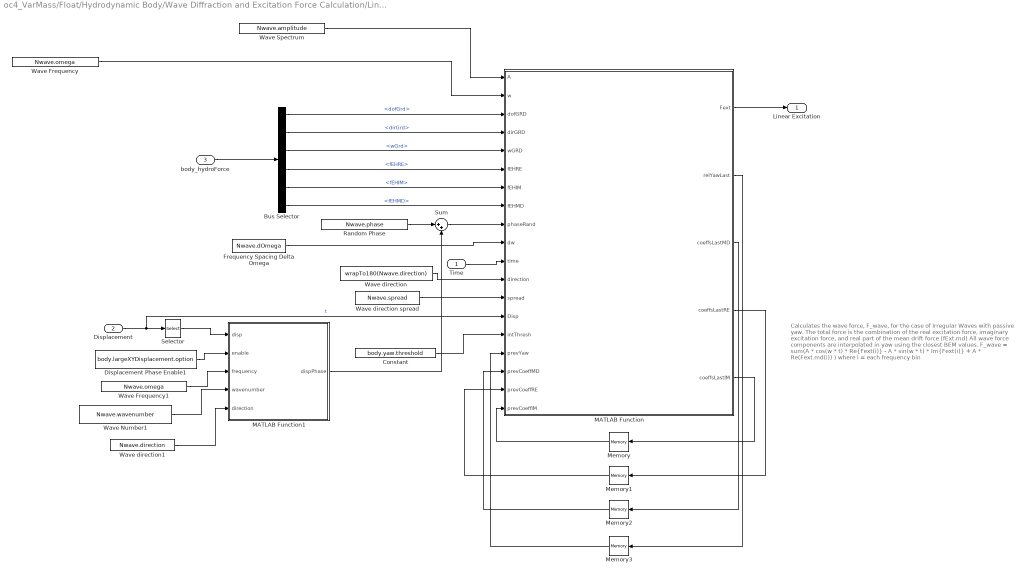
== system oc4_VarMass/Float/Hydrodynamic Body/Wave Diffraction and Excitation Force Calculation/Linear Wave Excitation Force Variant Subsystem/Irregular Wave NonLinearYaw ==
  note: Calculates the wave force, F_wave, for the case of Irregular Waves with passive yaw.
      |
      | The total force is the combination of the real excitation force, imaginary excitation force, and real part of the mean drift force (fExt.md)
      |
      | All wave force components are interpolated in yaw using the closest BEM values.
      |
      | F_wave =   sum(A * cos(w * t) * Re{Fext(i)}
      |                            -  A * sin(w * t) * Im{Fext(i)}
      |                            + A * Re(Fext.md(i))
      |                            )
      |
      | where i = each frequency bin
  Time : Inport
  Displacement : Inport  Port=2
  body_hydroForce : Inport  Port=3
  Bus Selector : BusSelector  OutputSignals=fExt.dofGrd,fExt.dirGrd,fExt.wGrd,fExt.fEHRE,fExt.fEHIM,fExt.fEHMD
  Constant : Constant  Value=body.yaw.threshold
  Displacement Phase Enable1 : Constant  Value=body.largeXYDisplacement.option
  Frequency Spacing Delta Omega : Constant  Value=Nwave.dOmega  VectorParams1D=off
  MATLAB Function : MATLAB Function  TreatAsAtomicUnit=on
  MATLAB Function1 : MATLAB Function  TreatAsAtomicUnit=on
  Memory{,1..3} (4 alike) : Memory  InheritSampleTime=on  LinearizeAsDelay=on
  Random Phase : Constant  Value=Nwave.phase  VectorParams1D=off
  Selector : Selector  IndexOptions=Index vector (dialog)  Indices=[1 2]  OutputSizes=1
  Sum : Sum  Inputs=|++
  Wave Frequency : Constant  Value=Nwave.omega  VectorParams1D=off
  Wave Frequency1 : Constant  Value=Nwave.omega  VectorParams1D=off
  Wave Number1 : Constant  Value=Nwave.wavenumber
  Wave Spectrum : Constant  Value=Nwave.amplitude  VectorParams1D=off
  Wave direction : Constant  Value=wrapTo180(Nwave.direction)  VectorParams1D=off
  Wave direction spread : Constant  Value=Nwave.spread  VectorParams1D=off
  Wave direction1 : Constant  Value=Nwave.direction  VectorParams1D=off
  Linear Excitation : Outport
  wires:
  Bus Selector/5 -> MATLAB Function/7(fEHIM)  "<fEHIM>"
  Bus Selector/1 -> MATLAB Function/3(dofGRD)  "<dofGrd>"
  body_hydroForce/1 -> Bus Selector/1
  MATLAB Function1/1(dispPhase) -> Sum/2
  Wave direction1/1 -> MATLAB Function1/5(direction)
  Wave Number1/1 -> MATLAB Function1/4(wavenumber)
  Displacement/1 -> Selector/1, MATLAB Function/14(Disp)  "t"
  Selector/1 -> MATLAB Function1/1(disp)
  Displacement Phase Enable1/1 -> MATLAB Function1/2(enable)
  Wave Frequency1/1 -> MATLAB Function1/3(frequency)
  Sum/1 -> MATLAB Function/9(phaseRand)
  Random Phase/1 -> Sum/1
  Time/1 -> MATLAB Function/11(time)
  Wave direction spread/1 -> MATLAB Function/13(spread)
  Bus Selector/6 -> MATLAB Function/8(fEHMD)  "<fEHMD>"
  Wave Spectrum/1 -> MATLAB Function/1(A)
  Wave Frequency/1 -> MATLAB Function/2(w)
  Memory/1 -> MATLAB Function/19(prevCoeffIM)
  Bus Selector/4 -> MATLAB Function/6(fEHRE)  "<fEHRE>"
  MATLAB Function/3(coeffsLastMD) -> Memory2/1
  Constant/1 -> MATLAB Function/15(intThresh)
  Memory3/1 -> MATLAB Function/16(prevYaw)
  MATLAB Function/5(coeffsLastIM) -> Memory/1
  Wave direction/1 -> MATLAB Function/12(direction)
  Frequency Spacing Delta Omega/1 -> MATLAB Function/10(dw)
  Bus Selector/2 -> MATLAB Function/4(dirGRD)  "<dirGrd>"
  Bus Selector/3 -> MATLAB Function/5(wGRD)  "<wGrd>"
  Memory2/1 -> MATLAB Function/17(prevCoeffMD)
  MATLAB Function/2(relYawLast) -> Memory3/1
  MATLAB Function/4(coeffsLastRE) -> Memory1/1
  Memory1/1 -> MATLAB Function/18(prevCoeffRE)
  MATLAB Function/1(Fext) -> Linear Excitation/1

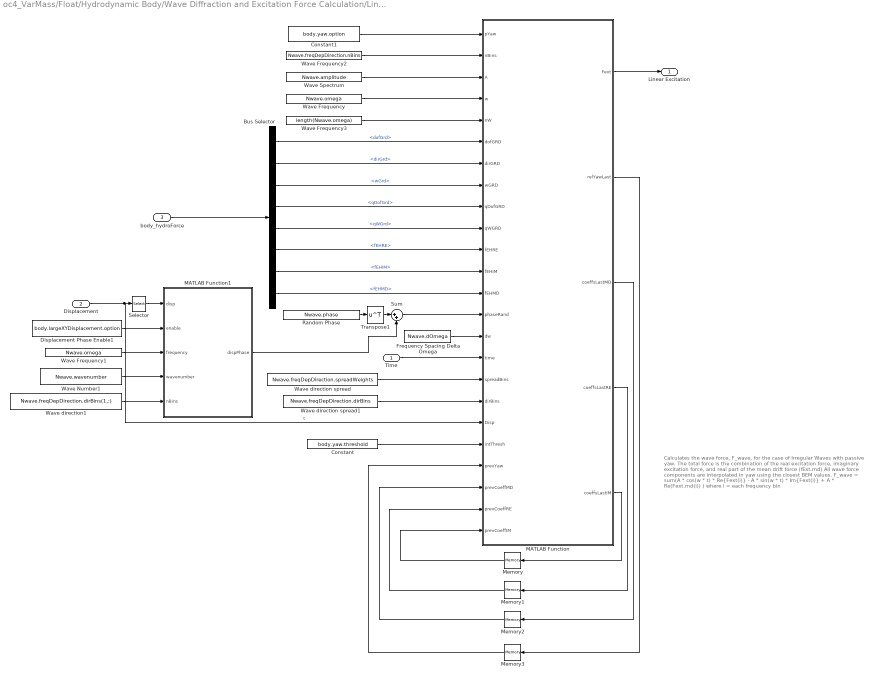
== system oc4_VarMass/Float/Hydrodynamic Body/Wave Diffraction and Excitation Force Calculation/Linear Wave Excitation Force Variant Subsystem/Irregular Wave Full Direction ==
  note: Calculates the wave force, F_wave, for the case of Irregular Waves with passive yaw.
      |
      | The total force is the combination of the real excitation force, imaginary excitation force, and real part of the mean drift force (fExt.md)
      |
      | All wave force components are interpolated in yaw using the closest BEM values.
      |
      | F_wave =   sum(A * cos(w * t) * Re{Fext(i)}
      |                            -  A * sin(w * t) * Im{Fext(i)}
      |                            + A * Re(Fext.md(i))
      |                            )
      |
      | where i = each frequency bin
  Time : Inport
  Displacement : Inport  Port=2
  body_hydroForce : Inport  Port=3
  Bus Selector : BusSelector  OutputSignals=fExt.dofGrd,fExt.dirGrd,fExt.wGrd,fExt.qDofGrd,fExt.qWGrd,fExt.fEHRE,fExt.fEHIM,fExt.fEHMD
  Constant : Constant  Value=body.yaw.threshold
  Constant1 : Constant  Value=body.yaw.option
  Displacement Phase Enable1 : Constant  Value=body.largeXYDisplacement.option
  Frequency Spacing Delta Omega : Constant  Value=Nwave.dOmega  VectorParams1D=off
  MATLAB Function : MATLAB Function  TreatAsAtomicUnit=on
  MATLAB Function1 : MATLAB Function  TreatAsAtomicUnit=on
  Memory : Memory  InitialCondition=zeros(Nwave.freqDepDirection.nBins,length(Nwave.omega),6)  InheritSampleTime=on  LinearizeAsDelay=on
  Memory1 : Memory  InitialCondition=zeros(Nwave.freqDepDirection.nBins,length(Nwave.omega),6)  InheritSampleTime=on  LinearizeAsDelay=on
  Memory2 : Memory  InitialCondition=zeros(Nwave.freqDepDirection.nBins,length(Nwave.omega),6)  InheritSampleTime=on  LinearizeAsDelay=on
  Memory3 : Memory  InitialCondition=zeros(length(Nwave.omega),Nwave.freqDepDirection.nBins)  InheritSampleTime=on  LinearizeAsDelay=on
  Random Phase : Constant  Value=Nwave.phase  VectorParams1D=off
  Selector : Selector  IndexOptions=Index vector (dialog)  Indices=[1 2]  OutputSizes=1
  Sum : Sum  Inputs=|++
  Transpose1 : Math  Operator=transpose
  Wave Frequency : Constant  Value=Nwave.omega  VectorParams1D=off
  Wave Frequency1 : Constant  Value=Nwave.omega  VectorParams1D=off
  Wave Frequency2 : Constant  Value=Nwave.freqDepDirection.nBins  VectorParams1D=off
  Wave Frequency3 : Constant  Value=length(Nwave.omega)  VectorParams1D=off
  Wave Number1 : Constant  Value=Nwave.wavenumber
  Wave Spectrum : Constant  Value=Nwave.amplitude  VectorParams1D=off
  Wave direction spread : Constant  Value=Nwave.freqDepDirection.spreadWeights  VectorParams1D=off
  Wave direction spread1 : Constant  Value=Nwave.freqDepDirection.dirBins  VectorParams1D=off
  Wave direction1 : Constant  Value=Nwave.freqDepDirection.dirBins(1,:)  VectorParams1D=off
  Linear Excitation : Outport
  wires:
  Transpose1/1 -> Sum/1
  MATLAB Function1/1(dispPhase) -> Sum/2
  Bus Selector/5 -> MATLAB Function/10(qWGRD)  "<qWGrd>"
  Bus Selector/4 -> MATLAB Function/9(qDofGRD)  "<qDofGrd>"
  Bus Selector/2 -> MATLAB Function/7(dirGRD)  "<dirGrd>"
  Bus Selector/8 -> MATLAB Function/13(fEHMD)  "<fEHMD>"
  Bus Selector/6 -> MATLAB Function/11(fEHRE)  "<fEHRE>"
  Bus Selector/1 -> MATLAB Function/6(dofGRD)  "<dofGrd>"
  body_hydroForce/1 -> Bus Selector/1
  Bus Selector/3 -> MATLAB Function/8(wGRD)  "<wGrd>"
  Bus Selector/7 -> MATLAB Function/12(fEHIM)  "<fEHIM>"
  Wave Frequency3/1 -> MATLAB Function/5(nW)
  Wave direction spread1/1 -> MATLAB Function/18(dirBins)
  MATLAB Function/2(relYawLast) -> Memory3/1
  Wave Number1/1 -> MATLAB Function1/4(wavenumber)
  Memory2/1 -> MATLAB Function/22(prevCoeffMD)
  Displacement/1 -> Selector/1, MATLAB Function/19(Disp)  "t"
  Memory3/1 -> MATLAB Function/21(prevYaw)
  Wave Frequency/1 -> MATLAB Function/4(w)
  Wave direction spread/1 -> MATLAB Function/17(spreadBins)
  Constant/1 -> MATLAB Function/20(intThresh)
  Time/1 -> MATLAB Function/16(time)
  MATLAB Function/5(coeffsLastIM) -> Memory/1
  Frequency Spacing Delta Omega/1 -> MATLAB Function/15(dw)
  Memory/1 -> MATLAB Function/24(prevCoeffIM)
  Memory1/1 -> MATLAB Function/23(prevCoeffRE)
  Wave Spectrum/1 -> MATLAB Function/3(A)
  Random Phase/1 -> Transpose1/1
  Sum/1 -> MATLAB Function/14(phaseRand)
  MATLAB Function/1(Fext) -> Linear Excitation/1
  Wave Frequency2/1 -> MATLAB Function/2(nBins)
  Wave Frequency1/1 -> MATLAB Function1/3(frequency)
  Selector/1 -> MATLAB Function1/1(disp)
  Displacement Phase Enable1/1 -> MATLAB Function1/2(enable)
  Wave direction1/1 -> MATLAB Function1/5(nBins)
  MATLAB Function/4(coeffsLastRE) -> Memory1/1
  MATLAB Function/3(coeffsLastMD) -> Memory2/1
  Constant1/1 -> MATLAB Function/1(pYaw)

== system oc4_VarMass/Float/Hydrodynamic Body/Wave Diffraction and Excitation Force Calculation/Linear Wave Excitation Force Variant Subsystem/No Wave Excitation Force ==
  Constant : Constant  Value=zeros(1,body.dof)
  Linear Excitation : Outport
  wires:
  Constant/1 -> Linear Excitation/1
